simulink subsystem "block_chain"  (R2025b)
settings: Solver=VariableStepAuto  StartTime=0.0  StopTime=10.0  RelTol=1e-3
settings Model: Creator=lenovo  LastModifiedBy=lenovo

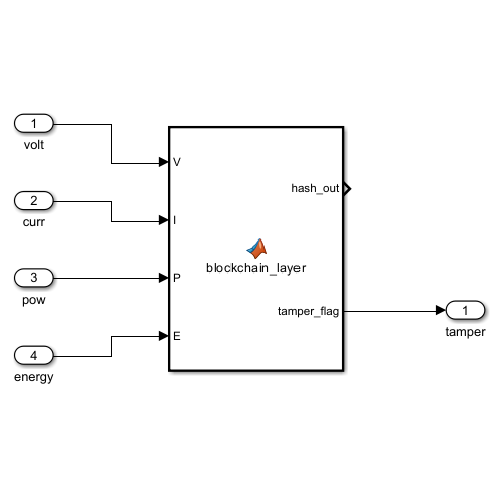
[thumbnail: Simulink's stored preview of the top-level diagram]
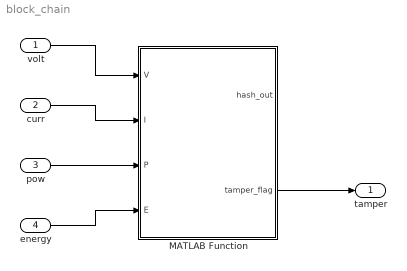
== system block_chain ==
  volt : Inport
  curr : Inport  Port=2
  pow : Inport  Port=3
  energy : Inport  Port=4
  MATLAB Function : MATLAB Function  TreatAsAtomicUnit=on
  tamper : Outport
  wires:
  volt/1 -> MATLAB Function/1(V)
  curr/1 -> MATLAB Function/2(I)
  pow/1 -> MATLAB Function/3(P)
  energy/1 -> MATLAB Function/4(E)
  MATLAB Function/2(tamper_flag) -> tamper/1

== matlab function block_chain/MATLAB Function ==
  data: V input; hash_out output; I input; P input; E input; tamper_flag output
function [hash_out, tamper_flag] = blockchain_layer(V, I, P, E)

persistent prev_hash

if isempty(prev_hash)
    prev_hash = 0;
end


current_hash = mod(abs(V*31 + I*17 + P*13 + E*7 + prev_hash), 1e6);

hash_out = current_hash;

if abs(current_hash - prev_hash) > 1e5
    tamper_flag = 1;
else
    tamper_flag = 0;
end

prev_hash = current_hash;

end
